simulink model "vishva_3"  (R2018b)
settings: Solver=VariableStepAuto  StartTime=0.0  StopTime=5  RelTol=1e-3
libraries: powerlib x12, simulink x2
settings Model: Creator=Admin  LastModifiedBy=Gokul

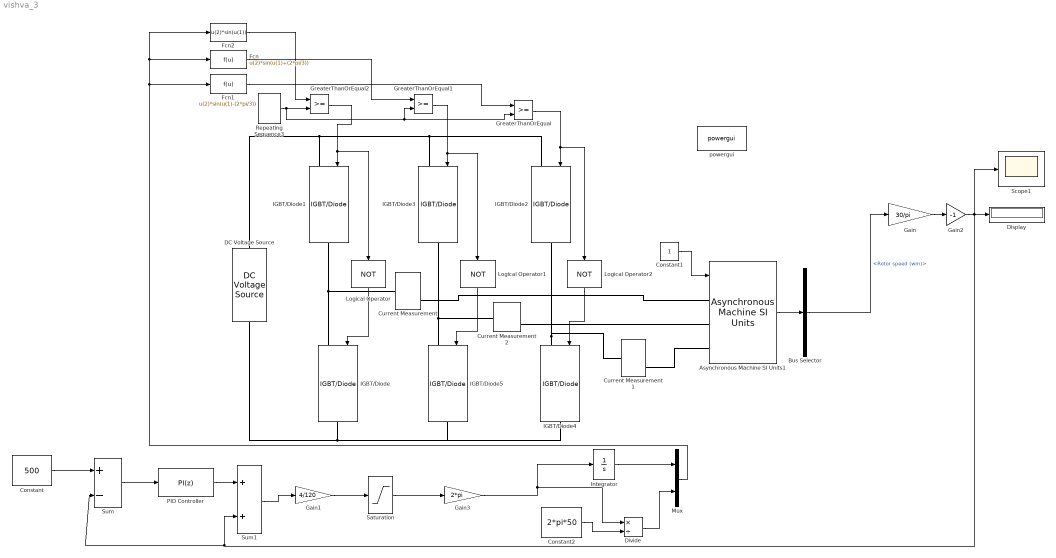
== system vishva_3 ==
  Asynchronous Machine SI Units1 : powerlib/Machines/Asynchronous Machine SI Units  RotorType=Squirrel-cage  PresetModel=No  MechanicalLoad=Torque Tm  ShowDetailedParameters=on  ReferenceFrame=Rotor  Units=SI  MeasurementBus=off  NominalParameters=[1.845e+04 400 50]  Stator=[0.5968 0.0003495]  Rotor=[0.6258 0.005473]  Cage1=[0.4155 0.002066]  Cage2=[0.4168 0.0003495]  Lm=0.0354  Mechanical=[0.05 0.005879 2]  PolePairs=2  InitialConditions=[1 0 0 0 0 0 0 0]  SimulateSaturation=off  Saturation=[14.03593122, 27.81365428, 53.79336849, 72.68890987, 97.98006896, 148.6815601, 215.7428561, 302.9841135, 428.7778367 ; 230, 322, 414, 460, 506, 552, 598, 644, 690]  LoadFlowParameters=1492000  TsPowergui=0  TsBlock=-1  IterativeModel=Trapezoidal non iterative  IterativeDiscreteModel=Trapezoidal non iterative  Pmec=1.492e+006
  Bus Selector : BusSelector  OutputSignals=Mechanical.Rotor speed (wm)
  Constant : Constant  Value=500
  Constant1 : Constant
  Constant2 : Constant  Value=2*pi*50
  Current Measurement : powerlib/Measurements/Current Measurement  PhasorSimulation=off  OutputType=Complex  PSBequivalent=0
  Current Measurement1 : powerlib/Measurements/Current Measurement  PhasorSimulation=off  OutputType=Complex  PSBequivalent=0
  Current Measurement2 : powerlib/Measurements/Current Measurement  PhasorSimulation=off  OutputType=Complex  PSBequivalent=0
  DC Voltage Source : powerlib/Electrical Sources/DC Voltage Source  Amplitude=650  Measurements=None
  Display : Display
  Divide : Product  Inputs=*/
  Fcn : Fcn  Expr=u(2)*sin(u(1)+(2*pi/3))
  Fcn1 : Fcn  Expr=u(2)*sin(u(1)-(2*pi/3))
  Fcn2 : Fcn  Expr=u(2)*sin(u(1))
  Gain : Gain  Gain=30/pi
  Gain1 : Gain  Gain=4/120
  Gain2 : Gain  Gain=-1
  Gain3 : Gain  Gain=2*pi
  GreaterThanOrEqual : RelationalOperator  OutDataTypeStr=boolean  RndMeth=Simplest
  GreaterThanOrEqual1 : RelationalOperator  OutDataTypeStr=boolean  RndMeth=Simplest
  GreaterThanOrEqual2 : RelationalOperator  OutDataTypeStr=boolean  RndMeth=Simplest
  IGBT/Diode{,1..5} (6 alike) : powerlib/Power Electronics/IGBT//Diode  Ron=1e-3  Rs=1e5  Cs=inf  Measurements=off
  Integrator : Integrator
  Logical Operator : Logic  Operator=NOT  AllPortsSameDT=off  OutDataTypeStr=boolean
  Logical Operator1 : Logic  Operator=NOT  AllPortsSameDT=off  OutDataTypeStr=boolean
  Logical Operator2 : Logic  Operator=NOT  AllPortsSameDT=off  OutDataTypeStr=boolean
  Mux : Mux  Inputs=2
  PID Controller : simulink/Continuous/PID Controller  Controller=PI  Form=Parallel  TimeDomain=Discrete-time  SampleTime=1e-5  IntegratorMethod=Forward Euler  FilterMethod=Forward Euler  ControllerParametersSource=internal  P=1  I=0.25  D=10  UseFilter=on  N=100  TunerSelectOption=Transfer Function Based (PID Tuner App)  InitialConditionSource=internal  InitialConditionForIntegrator=0  InitialConditionForFilter=0  DifferentiatorICPrevScaledInput=0  ExternalReset=none  TrackingMode=off  Kt=1  LimitOutput=on  UpperSaturationLimit=50  LowerSaturationLimit=-50  LinearizeAsGain=on  AntiWindupMode=clamping  Kb=1  POutMin=[]  POutMax=[]  IOutMin=[]  IOutMax=[]  DOutMin=[]  DOutMax=[]  NOutMin=[]  NOutMax=[]  SumOutMin=[]  SumOutMax=[]  SaturationOutMin=[]  SaturationOutMax=[]  PParamMin=[]  PParamMax=[]  IParamMin=[]  IParamMax=[]  DParamMin=[]  DParamMax=[]  NParamMin=[]  NParamMax=[]  KbParamMin=[]  KbParamMax=[]  KtParamMin=[]  KtParamMax=[]  KbOutMin=[]  KbOutMax=[]  KtOutMin=[]  KtOutMax=[]  IntegratorOutMin=[]  IntegratorOutMax=[]  FilterOutMin=[]  FilterOutMax=[]  SumI1OutMin=[]  SumI1OutMax=[]  SumI2OutMin=[]  SumI2OutMax=[]  SumI3OutMin=[]  SumI3OutMax=[]  SumI4OutMin=[]  SumI4OutMax=[]  SumDOutMin=[]  SumDOutMax=[]  DifferentiatorOutMin=[]  DifferentiatorOutMax=[]  FilterDiffOutCoefMin=[]  FilterDiffOutCoefMax=[]  ReciprocalOutMin=[]  ReciprocalOutMax=[]  SumDenOutMin=[]  SumDenOutMax=[]  SumNumOutMin=[]  SumNumOutMax=[]  DivideOutMin=[]  DivideOutMax=[]  IntegratorContinuousStateAttributes=''  IntegratorStateMustResolveToSignalObject=off  IntegratorRTWStateStorageClass=Auto  FilterContinuousStateAttributes=''  FilterStateMustResolveToSignalObject=off  FilterRTWStateStorageClass=Auto  ParallelPVariant=InternalParameters  IdealPVariant=Disabled  IVariant=InternalParameters  DVariant=Disabled  IntegratorVariant=Discrete  SatVariant=Enabled  AWVariant=DiscClampingParallel  PCopyVariant=Disabled  TRVariant=Disabled  FdbkBlocksVariant=Forward  IdealPFdbkVariant=Disabled  SatFdbkVariant=Disabled  DerivativeFilterVariant=Disabled  NVariant=Disabled  NCopyVariant=Disabled_SignalSpec  FilterICVariant=Disabled  IntegratorICVariant=InternalICs  ExternalResetVariant=Disabled  TRSumVariant=Passthrough  SumFdbkVariant=Disabled  SumVariant=Sum_PI
  Repeating Sequence3 : simulink/Sources/Repeating Sequence  rep_seq_t="[0   1   2]*1/5000"  rep_seq_y="[-1  1  -1]"
  Saturation : Saturate  UpperLimit=50  LowerLimit=0
  Scope1 : Scope
  Sum : Sum  Inputs=+-
  Sum1 : Sum
  powergui : powerlib/powergui  Priority=1  SimulationMode=Discrete  SampleTime=1e-6  frequency=60  Iterations=50  frequencyindice=50  Pbase=100e6  ErrMax=1e-4  UnitsV=kV  UnitsW=MW  buscounter=0  FunctionMessages=off  echomessages=off  EnableUseOfTLC=off  CurrentSourceSwitches=off  DisableSnubberDevices=off  DisableRonSwitches=off  DisableVfSwitches=off  DisplayEquations=off  SolverType=Tustin/Backward Euler (TBE)  Interpol=off  ExternalGateDelay=off  methode=off  Ts=100  x0status=blocks  SPID=on  SwTol=0  HookPort=off  RestoreLinks=warning  ResistiveCurrentMeasurement=off  Frange=[0:2:500]  Ylog=off  Xlog=on  ShowGrid=off  save=off  variable=ZData  structure=0  ZoomFFT=off  StartTime=0.0  cycles=1  DisplayStyle=1  fundamental=60  FreqAxis=off  MaxFrequency=1000  frequencyindicesteady=1  RmsSteady=1  display=off
  wires:
  Bus Selector/1 -> Gain/1  "<Rotor speed (wm)>"
  Fcn1/1 -> GreaterThanOrEqual/1
  Sum/1 -> PID Controller/1
  Sum1/1 -> Gain1/1
  Constant2/1 -> Divide/2
  Mux/1 -> Fcn2/1, Fcn/1, Fcn1/1
  Gain/1 -> Gain2/1
  Integrator/1 -> Mux/1
  Gain3/1 -> Divide/1, Integrator/1
  GreaterThanOrEqual2/1 -> Logical Operator/1, IGBT/Diode1/1
  Fcn2/1 -> GreaterThanOrEqual2/1
  Repeating Sequence3/1 -> GreaterThanOrEqual/2, GreaterThanOrEqual1/2, GreaterThanOrEqual2/2
  GreaterThanOrEqual1/1 -> Logical Operator1/1, IGBT/Diode3/1
  Constant/1 -> Sum/1
  Divide/1 -> Mux/2
  Gain1/1 -> Saturation/1
  Asynchronous Machine SI Units1/1 -> Bus Selector/1
  GreaterThanOrEqual/1 -> Logical Operator2/1, IGBT/Diode2/1
  Fcn/1 -> GreaterThanOrEqual1/1
  Logical Operator/1 -> IGBT/Diode/1
  Logical Operator2/1 -> IGBT/Diode4/1
  Gain2/1 -> Sum/2, Sum1/2, Display/1, Scope1/1
  Logical Operator1/1 -> IGBT/Diode5/1
  Constant1/1 -> Asynchronous Machine SI Units1/1
  PID Controller/1 -> Sum1/1
  Saturation/1 -> Gain3/1
  connections:
  IGBT/Diode4/LConn1 -- IGBT/Diode2/RConn1 -- Current Measurement1/LConn1
  IGBT/Diode/RConn1 -- DC Voltage Source/LConn1 -- IGBT/Diode4/RConn1 -- IGBT/Diode5/RConn1
  IGBT/Diode3/LConn1 -- IGBT/Diode1/LConn1 -- DC Voltage Source/RConn1 -- IGBT/Diode2/LConn1
  Current Measurement/LConn1 -- IGBT/Diode1/RConn1 -- IGBT/Diode/LConn1
  Current Measurement2/LConn1 -- IGBT/Diode3/RConn1 -- IGBT/Diode5/LConn1
  Current Measurement2/RConn1 -- Asynchronous Machine SI Units1/LConn2
  Current Measurement1/RConn1 -- Asynchronous Machine SI Units1/LConn3
  Current Measurement/RConn1 -- Asynchronous Machine SI Units1/LConn1
